simulink library "dynamicsLibrary"  (R2026a)
settings: Solver=ode45  EnableMultiTasking=on
undefined symbols (not defined in the file): Vehicle
libraries: sharedutil x2
settings Model: Creator=The MathWorks, Inc.  LastModifiedBy=The MathWorks, Inc.
settings DebuggingCC: UnderspecifiedInitializationDetection=Classic
settings HardwareCC: ProdHWDeviceType=32-bit Generic

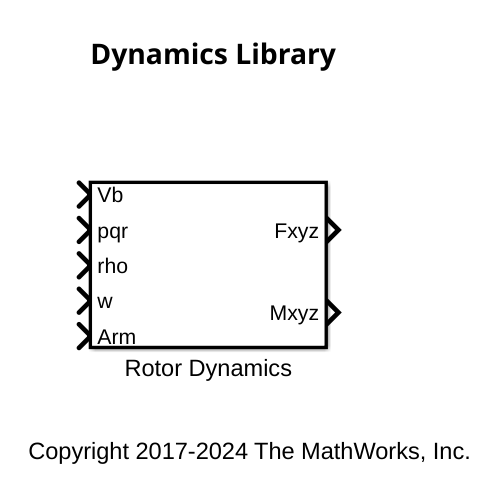
[thumbnail: Simulink's stored preview of the top-level diagram]
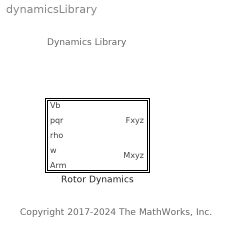
== system dynamicsLibrary ==
  note: Copyright 2017-2024 The MathWorks, Inc.
  note: Dynamics Library
  Rotor Dynamics : Subsystem  TreatAsAtomicUnit=on
      mask init:
      | aeroicon('aeroblk');
      settings: RTWFcnNameOpts=Use subsystem name  RTWFileNameOpts=Use function name

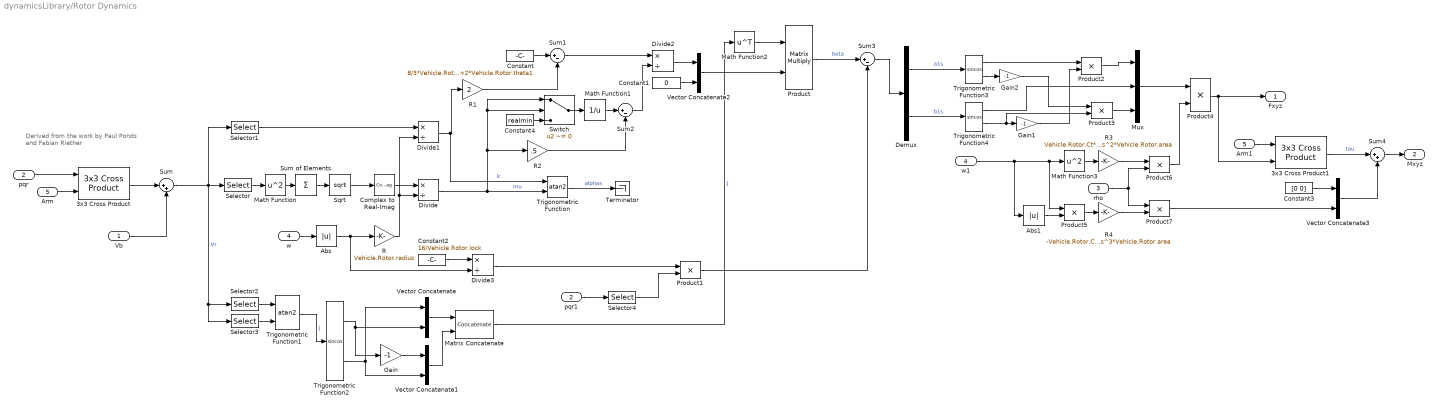
== system dynamicsLibrary/Rotor Dynamics ==
  note: Derived from the work by Paul Ponds
      | and Fabian Riether
  Vb : Inport  PortDimensions=3
  pqr : Inport  Port=2  PortDimensions=3
  rho : Inport  Port=3  PortDimensions=1
  w : Inport  Port=4  PortDimensions=[1 1]
  Arm : Inport  Port=5  PortDimensions=[3 1]
  3x3 Cross Product : sharedutil/3x3 Cross Product  aMode=aMode
  3x3 Cross Product1 : sharedutil/3x3 Cross Product  aMode=aMode
  Abs : Abs  SaturateOnIntegerOverflow=off
  Abs1 : Abs  SaturateOnIntegerOverflow=off
  Arm1 : InportShadow  Port=5  PortDimensions=[3 1]
  Complex to Real-Imag : ComplexToRealImag  Output=Real
  Constant : Constant  Value=8/3*Vehicle.Rotor.theta0+2*Vehicle.Rotor.theta1
  Constant1 : Constant  Value=0
  Constant2 : Constant  Value=16/Vehicle.Rotor.lock
  Constant3 : Constant  Value=[0 0]
  Constant4 : Constant  Value=realmin
  Demux : Demux  Outputs=2
  Divide{,1..3} (4 alike) : Product  Inputs=*/
  Gain : Gain  Gain=-1
  Gain1 : Gain  Gain=-1
  Gain2 : Gain  Gain=-1
  Math Function : Math  Operator=square  SignedPower=on
  Math Function1 : Math  Operator=reciprocal  SignedPower=on
  Math Function2 : Math  Operator=transpose  SignedPower=on
  Math Function3 : Math  Operator=square  SignedPower=on
  Matrix Concatenate : Concatenate  Mode=Multidimensional array  ConcatenateDimension=2
  Mux : Mux  Inputs=3
  Product : Product  Multiplication=Matrix(*)
  Product{1..7} (7 alike) : Product
  R : Gain  Gain=Vehicle.Rotor.radius
  R1 : Gain  Gain=2
  R2 : Gain  Gain=.5
  R3 : Gain  Gain=Vehicle.Rotor.Ct*Vehicle.Rotor.radius^2*Vehicle.Rotor.area
  R4 : Gain  Gain=-Vehicle.Rotor.Cq*Vehicle.Rotor.radius^3*Vehicle.Rotor.area
  Selector : Selector  InputPortWidth=3  IndexOptions=Index vector (dialog)  Indices=[1 2]  OutputSizes=1
  Selector1 : Selector  InputPortWidth=3  IndexOptions=Index vector (dialog)  Indices=[3]  OutputSizes=1
  Selector2 : Selector  InputPortWidth=3  IndexOptions=Index vector (dialog)  Indices=[2]  OutputSizes=1
  Selector3 : Selector  InputPortWidth=3  IndexOptions=Index vector (dialog)  Indices=[1]  OutputSizes=1
  Selector4 : Selector  InputPortWidth=3  IndexOptions=Index vector (dialog)  Indices=[2 1]  OutputSizes=1
  Sqrt : Sqrt  OutputSignalType=complex
  Sum : Sum  Inputs=|++
  Sum of Elements : Sum  Inputs=+
  Sum1 : Sum  Inputs=|+-
  Sum2 : Sum  Inputs=|+-
  Sum3 : Sum  Inputs=|+-
  Sum4 : Sum  Inputs=|++
  Switch : Switch  Criteria=u2 ~= 0  SaturateOnIntegerOverflow=off  InputSameDT=off
  Terminator : Terminator
  Trigonometric Function : Trigonometry  Operator=atan2
  Trigonometric Function1 : Trigonometry  Operator=atan2
  Trigonometric Function2 : Trigonometry  Operator=sincos
  Trigonometric Function3 : Trigonometry  Operator=sincos
  Trigonometric Function4 : Trigonometry  Operator=sincos
  Vector Concatenate{,1..3} (4 alike) : Concatenate
  pqr1 : InportShadow  Port=2  PortDimensions=3
  w1 : InportShadow  Port=4  PortDimensions=[1 1]
  Fxyz : Outport  PortDimensions=[3 1]  VectorParamsAs1DForOutWhenUnconnected=off
  Mxyz : Outport  Port=2  PortDimensions=[3 1]  VectorParamsAs1DForOutWhenUnconnected=off
  wires:
  3x3 Cross Product/1 -> Sum/1
  Vb/1 -> Sum/2
  Sum/1 -> Selector3/1, Selector2/1, Selector1/1, Selector/1  "Vr"
  Selector/1 -> Math Function/1
  Math Function/1 -> Sum of Elements/1
  Sum of Elements/1 -> Sqrt/1
  pqr/1 -> 3x3 Cross Product/1
  Arm/1 -> 3x3 Cross Product/2
  w/1 -> Abs/1
  R/1 -> Divide1/2, Divide/2
  Divide/1 -> R2/1, Switch/2, Switch/1, Trigonometric Function/2  "mu"
  Selector1/1 -> Divide1/1
  Divide1/1 -> R1/1, Trigonometric Function/1  "lc"
  Trigonometric Function/1 -> Terminator/1  "alphas"
  Selector2/1 -> Trigonometric Function1/1
  Selector3/1 -> Trigonometric Function1/2
  Trigonometric Function1/1 -> Trigonometric Function2/1  "j"
  Trigonometric Function2/2 -> Vector Concatenate1/2, Vector Concatenate/1
  Gain/1 -> Vector Concatenate1/1
  Trigonometric Function2/1 -> Vector Concatenate/2, Gain/1
  Vector Concatenate/1 -> Matrix Concatenate/1
  Vector Concatenate1/1 -> Matrix Concatenate/2
  Matrix Concatenate/1 -> Math Function2/1  "J"
  Constant/1 -> Sum1/1
  R1/1 -> Sum1/2
  Sum1/1 -> Divide2/1
  Math Function1/1 -> Sum2/1
  R2/1 -> Sum2/2
  Sum2/1 -> Divide2/2
  Divide2/1 -> Vector Concatenate2/1
  Constant1/1 -> Vector Concatenate2/2
  Vector Concatenate2/1 -> Product/2
  Math Function2/1 -> Product/1
  Product/1 -> Sum3/1  "beta"
  Constant2/1 -> Divide3/1
  pqr1/1 -> Selector4/1
  Selector4/1 -> Product1/2
  Abs/1 -> Divide3/2, R/1
  Divide3/1 -> Product1/1
  w1/1 -> Abs1/1, Product5/1, Math Function3/1
  Math Function3/1 -> R3/1
  Sum3/1 -> Demux/1
  Demux/1 -> Trigonometric Function3/1  "a1s"
  Demux/2 -> Trigonometric Function4/1  "b1s"
  Trigonometric Function4/2 -> Product3/2, Gain1/1
  Gain1/1 -> Product2/2
  Trigonometric Function3/1 -> Product2/1
  Product2/1 -> Mux/1
  Trigonometric Function4/1 -> Mux/2
  Trigonometric Function3/2 -> Gain2/1
  Product3/1 -> Mux/3
  Gain2/1 -> Product3/1
  Mux/1 -> Product4/1
  R3/1 -> Product6/1
  Abs1/1 -> Product5/2
  Product5/1 -> R4/1
  R4/1 -> Product7/2
  Constant3/1 -> Vector Concatenate3/1
  Vector Concatenate3/1 -> Sum4/2
  Arm1/1 -> 3x3 Cross Product1/1
  Product4/1 -> 3x3 Cross Product1/2, Fxyz/1
  3x3 Cross Product1/1 -> Sum4/1  "tau"
  Sum4/1 -> Mxyz/1
  Product6/1 -> Product4/2
  Product7/1 -> Vector Concatenate3/2
  rho/1 -> Product6/2, Product7/1
  Product1/1 -> Sum3/2
  Switch/1 -> Math Function1/1
  Constant4/1 -> Switch/3
  Sqrt/1 -> Complex to Real-Imag/1
  Complex to Real-Imag/1 -> Divide/1
